simulink model "im_inv_model"  (R2026a)
settings: Solver=ode23tb  StopTime=param.sim.simlength  FixedStep=param.sim.tc  MaxStep=param.glb_time.tc  EnableMultiTasking=on
values from neighbouring files (symbols this model uses):
  param = struct()    [init_model.m]
undefined symbols (not defined in the file or in its folder): magnitude
libraries: fl_lib x53, nesl_utility x25, simulink x2, lithium_ion_battery x1, induction_machine x1, threephase_inductor_lib x1, dclink_with_center_tap x1, cstblocks_lti x1
(part 3 of 3)

== system im_inv_model/inverter//ctrl/im_ctrl/im_control/current control/bounder1 ==
  md : Inport
  k_sat : Inport  Port=2
  m : Inport  Port=3
  Constant : Constant
  Constant1 : Constant  Value=0
  Divide : Product
  Switch : Switch  Threshold=sqrt(3)/2  SaturateOnIntegerOverflow=off  InputSameDT=off
  Switch1 : Switch  Threshold=1 %sqrt(3)/2  SaturateOnIntegerOverflow=off  InputSameDT=off
  md_sat : Outport  VectorParamsAs1DForOutWhenUnconnected=off
  clip : Outport  Port=2  VectorParamsAs1DForOutWhenUnconnected=off
  wires:
  md/1 -> Switch1/3, Divide/2
  k_sat/1 -> Divide/1
  Divide/1 -> Switch1/1
  Switch1/1 -> md_sat/1
  Switch/1 -> clip/1
  m/1 -> Switch/2, Switch1/2
  Constant/1 -> Switch/1
  Constant1/1 -> Switch/3

== system im_inv_model/inverter//ctrl/im_ctrl/im_control/current control/bounder2 ==
  m : Inport
  k_sat : Inport  Port=2
  mq : Inport  Port=3
  Constant : Constant
  Constant1 : Constant  Value=0
  Divide : Product
  Switch : Switch  Threshold=sqrt(3)/2  SaturateOnIntegerOverflow=off  InputSameDT=off
  Switch1 : Switch  Threshold=1 %sqrt(3)/2  SaturateOnIntegerOverflow=off  InputSameDT=off
  mq_sat : Outport  VectorParamsAs1DForOutWhenUnconnected=off
  clip : Outport  Port=2  VectorParamsAs1DForOutWhenUnconnected=off
  wires:
  Constant1/1 -> Switch/3
  Constant/1 -> Switch/1
  m/1 -> Switch1/2, Switch/2
  Switch/1 -> clip/1
  Switch1/1 -> mq_sat/1
  Divide/1 -> Switch1/1
  k_sat/1 -> Divide/1
  mq/1 -> Divide/2, Switch1/3

== system im_inv_model/inverter//ctrl/im_ctrl/im_control/current control/pi-ctrl-x ==
  id_tilde : Inport
  clip : Inport  Port=2
  1/Ti : Gain  Gain=param.im.ctrl.kp_inv_d  SaturateOnIntegerOverflow=on  OutDataTypeStr=Inherit: Same as input  ParamDataTypeStr=Inherit: Same as input
  Constant : Constant  Value=0
  Sum2 : Sum  Inputs=+-  SaturateOnIntegerOverflow=on
  Sum4 : Sum  SaturateOnIntegerOverflow=on
  Sum5 : Sum  SaturateOnIntegerOverflow=on
  Switch1 : Switch  Threshold=0.5  SaturateOnIntegerOverflow=off  InputSameDT=off
  Switch2 : Switch  Threshold=0.5  SaturateOnIntegerOverflow=off  InputSameDT=off
  Unit Delay1 : UnitDelay  SampleTime=param.glb_time.ts_inv
  Unit Delay2 : UnitDelay  SampleTime=param.glb_time.ts_inv
  kp1 : Gain  Gain=param.ctrl.CTRPIFF_CLIP_RELEASE*param.glb_time.ts_inv  SaturateOnIntegerOverflow=on  OutDataTypeStr=Inherit: Same as input  ParamDataTypeStr=Inherit: Same as input
  kp2 : Gain  Gain=param.im.ctrl.ki_inv_d*param.glb_time.ts_inv  SaturateOnIntegerOverflow=on  OutDataTypeStr=Inherit: Same as input  ParamDataTypeStr=Inherit: Same as input
  Vds_out : Outport  VectorParamsAs1DForOutWhenUnconnected=off
  wires:
  id_tilde/1 -> kp2/1, 1/Ti/1
  Sum5/1 -> Vds_out/1
  Switch1/1 -> Unit Delay2/1
  Sum4/1 -> Sum5/2, Switch1/3
  kp1/1 -> Sum2/2
  Sum2/1 -> Switch1/1
  Unit Delay2/1 -> Sum4/2, kp1/1, Sum2/1
  1/Ti/1 -> Sum5/1
  Switch2/1 -> Sum4/1
  kp2/1 -> Switch2/3
  clip/1 -> Unit Delay1/1
  [clip] -> Switch2/2
  [clip] -> Switch1/2
  Constant/1 -> Switch2/1
  Unit Delay1/1 -> [clip]

== system im_inv_model/inverter//ctrl/im_ctrl/im_control/current control/pi-ctrl-y ==
  iq_tilde : Inport
  clip : Inport  Port=2
  1/Ti : Gain  Gain=param.im.ctrl.kp_inv_q  SaturateOnIntegerOverflow=on  OutDataTypeStr=Inherit: Same as input  ParamDataTypeStr=Inherit: Same as input
  Constant : Constant  Value=0
  Sum2 : Sum  Inputs=+-  SaturateOnIntegerOverflow=on
  Sum4 : Sum  SaturateOnIntegerOverflow=on
  Sum5 : Sum  SaturateOnIntegerOverflow=on
  Switch1 : Switch  Threshold=0.5  SaturateOnIntegerOverflow=off  InputSameDT=off
  Switch2 : Switch  Threshold=0.5  SaturateOnIntegerOverflow=off  InputSameDT=off
  Unit Delay1 : UnitDelay  SampleTime=param.glb_time.ts_inv
  Unit Delay2 : UnitDelay  SampleTime=param.glb_time.ts_inv
  kp1 : Gain  Gain=param.ctrl.CTRPIFF_CLIP_RELEASE*param.glb_time.ts_inv  SaturateOnIntegerOverflow=on  OutDataTypeStr=Inherit: Same as input  ParamDataTypeStr=Inherit: Same as input
  kp2 : Gain  Gain=param.im.ctrl.ki_inv_q*param.glb_time.ts_inv  SaturateOnIntegerOverflow=on  OutDataTypeStr=Inherit: Same as input  ParamDataTypeStr=Inherit: Same as input
  Vqs_out : Outport  VectorParamsAs1DForOutWhenUnconnected=off
  wires:
  Constant/1 -> Switch2/1
  [clip] -> Switch1/2
  [clip] -> Switch2/2
  clip/1 -> Unit Delay1/1
  kp2/1 -> Switch2/3
  Switch2/1 -> Sum4/1
  1/Ti/1 -> Sum5/1
  Unit Delay2/1 -> Sum2/1, kp1/1, Sum4/2
  Sum2/1 -> Switch1/1
  kp1/1 -> Sum2/2
  Sum4/1 -> Sum5/2, Switch1/3
  Switch1/1 -> Unit Delay2/1
  Sum5/1 -> Vqs_out/1
  iq_tilde/1 -> 1/Ti/1, kp2/1
  Unit Delay1/1 -> [clip]

== system im_inv_model/inverter//ctrl/im_ctrl/im_control/current control/switch ==
  clip 1 : Inport
  clip 2 : Inport  Port=2
  Constant4 : Constant
  Constant5 : Constant  Value=0
  Sum1 : Sum  SaturateOnIntegerOverflow=on
  Switch : Switch  Threshold=0.5  SaturateOnIntegerOverflow=off  InputSameDT=off
  clip : Outport  VectorParamsAs1DForOutWhenUnconnected=off
  wires:
  Constant5/1 -> Switch/3
  Switch/1 -> clip/1
  Constant4/1 -> Switch/1
  Sum1/1 -> Switch/2
  clip 1/1 -> Sum1/1
  clip 2/1 -> Sum1/2

== system im_inv_model/inverter//ctrl/im_ctrl/im_control/current control/vector lenght ==
  md : Inport
  mq : Inport  Port=2
  1/Ti3 : Gain  Gain=sqrt(3)/2  SaturateOnIntegerOverflow=on  OutDataTypeStr=Inherit: Same as input  ParamDataTypeStr=Inherit: Same as input
  Math Function : Math  Operator=magnitude^2  SignedPower=on
  Math Function1 : Math  Operator=magnitude^2  SignedPower=on
  Math Function2 : Math  Operator=reciprocal  SignedPower=on
  Sqrt : Sqrt
  Sum5 : Sum  SaturateOnIntegerOverflow=on
  k_sat : Outport  VectorParamsAs1DForOutWhenUnconnected=off
  m : Outport  Port=2  VectorParamsAs1DForOutWhenUnconnected=off
  wires:
  Sqrt/1 -> m/1, Math Function2/1
  mq/1 -> Math Function1/1
  Math Function1/1 -> Sum5/2
  Math Function/1 -> Sum5/1
  Sum5/1 -> Sqrt/1
  Math Function2/1 -> k_sat/1
  md/1 -> Math Function/1

== system im_inv_model/inverter//ctrl/im_ctrl/im_control/data_analysis/double_integrator_observer_1 ==
  theta : Inport
  Gain : Gain  Gain=param.im.ctrl.di_obs.komega
  Gain1 : Gain  Gain=param.im.ctrl.di_obs.ktheta
  Gain2 : Gain  Gain=param.im.machine.omega_bez
  Gain3 : Gain  Gain=1/param.im.machine.omega_bez
  Gain5 : Gain  Gain=param.glb_time.ts_inv
  Sum : Sum  Inputs=-+|
  Sum1 : Sum  Inputs=|++
  Sum2 : Sum  Inputs=|++
  Sum8 : Sum  Inputs=++|
  Unit Delay1 : UnitDelay  InitialCondition=pi  SampleTime=param.glb_time.ts_inv
  Unit Delay2 : UnitDelay  SampleTime=param.glb_time.ts_inv
  bounder1 : MATLAB Function  TreatAsAtomicUnit=on  SystemSampleTime=param.glb_time.ts_inv
  bounder2 : MATLAB Function  TreatAsAtomicUnit=on  SystemSampleTime=param.glb_time.ts_inv
  omega_pu_hat : Outport  VectorParamsAs1DForOutWhenUnconnected=off
  wires:
  Gain1/1 -> Sum2/1
  theta/1 -> Sum/2  "theta_bemf"
  Sum8/1 -> Unit Delay1/1
  Unit Delay1/1 -> bounder2/1(u)
  Sum1/1 -> Unit Delay2/1
  Gain/1 -> Gain3/1
  Unit Delay2/1 -> omega_pu_hat/1, Sum1/2, Gain5/1
  Sum2/1 -> Sum8/2
  bounder2/1(y) -> Sum2/2, Sum/1  "theta_hat"
  bounder1/1(y) -> Gain1/1, Gain/1
  Gain2/1 -> Sum8/1
  Gain3/1 -> Sum1/1
  Gain5/1 -> Gain2/1
  Sum/1 -> bounder1/1(u)

== system im_inv_model/inverter//ctrl/im_ctrl/im_control/data_analysis/double_integrator_observer_2 ==
  theta : Inport
  Gain : Gain  Gain=param.im.ctrl.di_obs.komega
  Gain1 : Gain  Gain=param.im.ctrl.di_obs.ktheta
  Gain2 : Gain  Gain=param.im.machine.omega_bez
  Gain3 : Gain  Gain=1/param.im.machine.omega_bez
  Gain5 : Gain  Gain=param.glb_time.ts_inv
  Sum : Sum  Inputs=-+|
  Sum1 : Sum  Inputs=|++
  Sum2 : Sum  Inputs=|++
  Sum8 : Sum  Inputs=++|
  Unit Delay1 : UnitDelay  InitialCondition=pi  SampleTime=param.glb_time.ts_inv
  Unit Delay2 : UnitDelay  SampleTime=param.glb_time.ts_inv
  bounder1 : MATLAB Function  TreatAsAtomicUnit=on  SystemSampleTime=param.glb_time.ts_inv
  bounder2 : MATLAB Function  TreatAsAtomicUnit=on  SystemSampleTime=param.glb_time.ts_inv
  omega_pu_hat : Outport  VectorParamsAs1DForOutWhenUnconnected=off
  wires:
  Sum/1 -> bounder1/1(u)
  Gain5/1 -> Gain2/1
  Gain3/1 -> Sum1/1
  Gain2/1 -> Sum8/1
  bounder1/1(y) -> Gain/1, Gain1/1
  bounder2/1(y) -> Sum/1, Sum2/2  "theta_hat"
  Sum2/1 -> Sum8/2
  Unit Delay2/1 -> Gain5/1, Sum1/2, omega_pu_hat/1
  Gain/1 -> Gain3/1
  Sum1/1 -> Unit Delay2/1
  Unit Delay1/1 -> bounder2/1(u)
  Sum8/1 -> Unit Delay1/1
  theta/1 -> Sum/2  "theta_bemf"
  Gain1/1 -> Sum2/1

== system im_inv_model/inverter//ctrl/im_ctrl/im_control/data_analysis/double_integrator_observer_3 ==
  theta : Inport
  Gain : Gain  Gain=param.im.ctrl.di_obs.komega
  Gain1 : Gain  Gain=param.im.ctrl.di_obs.ktheta
  Gain2 : Gain  Gain=param.im.machine.omega_bez
  Gain3 : Gain  Gain=1/param.im.machine.omega_bez
  Gain5 : Gain  Gain=param.glb_time.ts_inv
  Sum : Sum  Inputs=-+|
  Sum1 : Sum  Inputs=|++
  Sum2 : Sum  Inputs=|++
  Sum8 : Sum  Inputs=++|
  Unit Delay1 : UnitDelay  InitialCondition=pi  SampleTime=param.glb_time.ts_inv
  Unit Delay2 : UnitDelay  SampleTime=param.glb_time.ts_inv
  bounder1 : MATLAB Function  TreatAsAtomicUnit=on  SystemSampleTime=param.glb_time.ts_inv
  bounder2 : MATLAB Function  TreatAsAtomicUnit=on  SystemSampleTime=param.glb_time.ts_inv
  omega_pu_hat : Outport  VectorParamsAs1DForOutWhenUnconnected=off
  wires:
  Gain1/1 -> Sum2/1
  theta/1 -> Sum/2  "theta_bemf"
  Sum8/1 -> Unit Delay1/1
  Unit Delay1/1 -> bounder2/1(u)
  Sum1/1 -> Unit Delay2/1
  Gain/1 -> Gain3/1
  Unit Delay2/1 -> omega_pu_hat/1, Sum1/2, Gain5/1
  Sum2/1 -> Sum8/2
  bounder2/1(y) -> Sum2/2, Sum/1  "theta_hat"
  bounder1/1(y) -> Gain1/1, Gain/1
  Gain2/1 -> Sum8/1
  Gain3/1 -> Sum1/1
  Gain5/1 -> Gain2/1
  Sum/1 -> bounder1/1(u)

== system im_inv_model/inverter//ctrl/im_ctrl/im_control/flux_estimator/alphabeta2dq ==
  alpha : Inport
  beta : Inport  Port=2
  phase : Inport  Port=3
  Gain : Gain
  Gain1 : Gain
  Product{,1..3} (4 alike) : Product  RndMeth=Zero
  Sum : Sum
  Sum1 : Sum  Inputs=-+
  Trigonometric Function : Trigonometry  Operator=cos
  Trigonometric Function1 : Trigonometry
  d : Outport  VectorParamsAs1DForOutWhenUnconnected=off
  q : Outport  Port=2  VectorParamsAs1DForOutWhenUnconnected=off
  wires:
  [cos] -> Product/1
  alpha/1 -> Product/2, Product2/2
  Product/1 -> Sum/1
  Product1/1 -> Sum/2
  [sin] -> Product1/1
  beta/1 -> Product1/2, Product3/2
  Sum/1 -> Gain/1
  [sin] -> Product2/1
  Product2/1 -> Sum1/1
  Product3/1 -> Sum1/2
  [cos] -> Product3/1
  Sum1/1 -> Gain1/1
  Gain/1 -> d/1
  Gain1/1 -> q/1
  Trigonometric Function1/1 -> [sin]
  Trigonometric Function/1 -> [cos]
  phase/1 -> Trigonometric Function/1, Trigonometric Function1/1

== system im_inv_model/inverter//ctrl/im_ctrl/im_control/magnetization current reference/pi ==
  psi_r_hat : Inport
  psi_r_ref : Inport  Port=2
  1/Ti : Gain  Gain=param.im.ctrl.kp_psi  SaturateOnIntegerOverflow=on  OutDataTypeStr=Inherit: Same as input  ParamDataTypeStr=Inherit: Same as input
  Saturation : Saturate  UpperLimit=param.im.ctrl.isx_lim_max*param.im.machine.Lm_norm  LowerLimit=param.im.ctrl.isx_lim_min*param.im.machine.Lm_norm
  Sum1 : Sum  Inputs=+++  SaturateOnIntegerOverflow=on
  Sum2 : Sum  Inputs=-+  SaturateOnIntegerOverflow=on
  Sum3 : Sum  Inputs=-+  SaturateOnIntegerOverflow=on
  Unit Delay4 : UnitDelay  SampleTime=param.glb_time.ts_inv
  kp : Gain  Gain=param.im.ctrl.ki_psi*param.glb_time.ts_inv  SaturateOnIntegerOverflow=on  OutDataTypeStr=Inherit: Same as input  ParamDataTypeStr=Inherit: Same as input
  psi_s_ref : Outport  VectorParamsAs1DForOutWhenUnconnected=off
  wires:
  1/Ti/1 -> Sum1/1, Sum3/1
  kp/1 -> Sum1/2
  Sum2/1 -> 1/Ti/1, kp/1
  Sum1/1 -> Saturation/1
  Sum3/1 -> Unit Delay4/1
  Unit Delay4/1 -> Sum1/3
  psi_r_ref/1 -> Sum2/2
  psi_r_hat/1 -> Sum2/1
  Saturation/1 -> psi_s_ref/1, Sum3/2

== system im_inv_model/inverter//ctrl/im_ctrl/im_control/u//f control/uf_phase_generation ==
  Constant1 : Constant  Value=param.im.uf.omega_ref
  Gain : Gain  Gain=param.im.uf.Omega_s_bez
  Integrator : Integrator
  Zero-Order Hold : ZeroOrderHold  SampleTime=param.glb_time.ts_inv
  bounder : MATLAB Function  TreatAsAtomicUnit=on  SystemSampleTime=param.glb_time.ts_inv
  uf_electrical_phase : Outport
  wires:
  Gain/1 -> Integrator/1
  Integrator/1 -> Zero-Order Hold/1
  Zero-Order Hold/1 -> bounder/1(u)
  Constant1/1 -> Gain/1
  bounder/1(y) -> uf_electrical_phase/1

== system im_inv_model/inverter//ctrl/inverter/inverter/sv_pwm/modulator1 ==
  u : Inport
  v : Inport  Port=2
  w : Inport  Port=3
  phase : Inport  Port=4
  Bus Creator3 : BusCreator  Inputs=6
  PWM generator 1 : Subsystem  mask{f=param.glb_time.fPWM_INV, m_up=0.98, m_low=0.02, dead_time=param.glb_time.dead_time_INV, pos_cmd_gate=15, neg_cmd_gate=-10, polarity=-1}
      mask prompts: f "Frequency (Hz)"; m_up "Max Input Modulation Value"; m_low "Min Input Modulation Value"; dead_time "Dead Time (s)"; pos_cmd_gate "Positive Gate Voltage (V)"; neg_cmd_gate "Negative Gate Voltage (V)"; polarity "Polarity (pu)"
  PWM generator 2 : Subsystem  mask{f=param.glb_time.fPWM_INV, m_up=0.98, m_low=0.02, dead_time=param.glb_time.dead_time_INV, pos_cmd_gate=15, neg_cmd_gate=-10, polarity=-1}
      mask prompts: f "Frequency (Hz)"; m_up "Max Input Modulation Value"; m_low "Min Input Modulation Value"; dead_time "Dead Time (s)"; pos_cmd_gate "Positive Gate Voltage (V)"; neg_cmd_gate "Negative Gate Voltage (V)"; polarity "Polarity (pu)"
  PWM generator 3 : Subsystem  mask{f=param.glb_time.fPWM_INV, m_up=0.98, m_low=0.02, dead_time=param.glb_time.dead_time_INV, pos_cmd_gate=15, neg_cmd_gate=-10, polarity=-1}
      mask prompts: f "Frequency (Hz)"; m_up "Max Input Modulation Value"; m_low "Min Input Modulation Value"; dead_time "Dead Time (s)"; pos_cmd_gate "Positive Gate Voltage (V)"; neg_cmd_gate "Negative Gate Voltage (V)"; polarity "Polarity (pu)"
  cmd_gates : Outport
  wires:
  u/1 -> PWM generator 1/1(m_index)
  w/1 -> PWM generator 3/1(m_index)
  v/1 -> PWM generator 2/1(m_index)
  phase/1 -> PWM generator 3/2(phase), PWM generator 2/2(phase), PWM generator 1/2(phase)
  PWM generator 1/2(m2) -> Bus Creator3/2  "gate_cmd_Q2"
  PWM generator 3/1(m1) -> Bus Creator3/5  "gate_cmd_Q5"
  PWM generator 2/1(m1) -> Bus Creator3/3  "gate_cmd_Q3"
  PWM generator 2/2(m2) -> Bus Creator3/4  "gate_cmd_Q4"
  PWM generator 3/2(m2) -> Bus Creator3/6  "gate_cmd_Q6"
  PWM generator 1/1(m1) -> Bus Creator3/1  "gate_cmd_Q1"
  Bus Creator3/1 -> cmd_gates/1

== system im_inv_model/inverter//ctrl/inverter/inverter/three phase pwm/Third harmonic injecting ==
  m1 : Inport
  m2 : Inport  Port=2
  m3 : Inport  Port=3
  Gain : Gain  Gain=1/2
  MinMax : MinMax  Function=max  Inputs=3
  MinMax1 : MinMax  Inputs=3
  Sum : Sum  Inputs=|++
  trn : Outport
  wires:
  Gain/1 -> trn/1
  Sum/1 -> Gain/1
  MinMax1/1 -> Sum/2
  MinMax/1 -> Sum/1
  m3/1 -> MinMax/3, MinMax1/3
  m1/1 -> MinMax1/1, MinMax/1
  m2/1 -> MinMax1/2, MinMax/2

== system im_inv_model/inverter//ctrl/inverter/inverter/three phase pwm/modulator ==
  u : Inport
  v : Inport  Port=2
  w : Inport  Port=3
  phase : Inport  Port=4
  Bus Creator3 : BusCreator  Inputs=6
  PWM generator 1 : Subsystem  mask{f=param.glb_time.fPWM_INV, m_up=1, m_low=0, dead_time=0, vg_firing=15}
      mask prompts: f "Frequency"; m_up "Max Input Modulation Value"; m_low "Min Input Modulation Value"; dead_time "Dead Time"; vg_firing "Gate Voltage"
  PWM generator 2 : Subsystem  mask{f=param.glb_time.fPWM_INV, m_up=1, m_low=0, dead_time=0, vg_firing=15}
      mask prompts: f "Frequency"; m_up "Max Input Modulation Value"; m_low "Min Input Modulation Value"; dead_time "Dead Time"; vg_firing "Gate Voltage"
  PWM generator 3 : Subsystem  mask{f=param.glb_time.fPWM_INV, m_up=1, m_low=0, dead_time=0, vg_firing=15}
      mask prompts: f "Frequency"; m_up "Max Input Modulation Value"; m_low "Min Input Modulation Value"; dead_time "Dead Time"; vg_firing "Gate Voltage"
  cmd_gates : Outport
  wires:
  u/1 -> PWM generator 1/1(m_index)
  w/1 -> PWM generator 3/1(m_index)
  v/1 -> PWM generator 2/1(m_index)
  phase/1 -> PWM generator 3/2(phase), PWM generator 2/2(phase), PWM generator 1/2(phase)
  PWM generator 3/2(m2) -> Bus Creator3/6  "gate_cmd_Q6"
  Bus Creator3/1 -> cmd_gates/1
  PWM generator 2/2(m2) -> Bus Creator3/4  "gate_cmd_Q4"
  PWM generator 1/1(m1) -> Bus Creator3/1  "gate_cmd_Q1"
  PWM generator 3/1(m1) -> Bus Creator3/5  "gate_cmd_Q5"
  PWM generator 1/2(m2) -> Bus Creator3/2  "gate_cmd_Q2"
  PWM generator 2/1(m1) -> Bus Creator3/3  "gate_cmd_Q3"

== system im_inv_model/inverter//ctrl/inverter/inverter/three phase pwm1/PWM generator 1 ==
  m_index : Inport
  Constant : Constant  Value=dead_time*f*2
  Data Type Conversion1 : DataTypeConversion
  Data Type Conversion2 : DataTypeConversion
  Gain : Gain  Gain=1/(pi/2)
  Gain1 : Gain  Gain=sqrt(3)/2
  Hit Crossing : HitCross  ShowOutputPort=off
  Hit Crossing1 : HitCross  ShowOutputPort=off
  Relational Operator1 : RelationalOperator  Operator=<=  InputSameDT=off
  Relational Operator2 : RelationalOperator  Operator=<=  InputSameDT=off
  Saturation1 : Saturate  UpperLimit=m_up  LowerLimit=m_low
  Sine Wave : Sin  Frequency=f*2*pi  Phase=-pi/2+ph  SampleTime=0
  Sum : Sum  Inputs=|++  SaturateOnIntegerOverflow=on
  Sum1 : Sum  Inputs=-+|  SaturateOnIntegerOverflow=on
  Trigonometric Function1 : Trigonometry  Operator=asin
  m1 : Outport
  m2 : Outport  Port=2
  wires:
  Relational Operator1/1 -> Data Type Conversion1/1
  m_index/1 -> Saturation1/1
  Data Type Conversion1/1 -> Hit Crossing/1, m2/1
  Relational Operator2/1 -> Data Type Conversion2/1
  Data Type Conversion2/1 -> Hit Crossing1/1, m1/1
  Constant/1 -> Sum/2, Sum1/1
  Saturation1/1 -> Sum/1, Sum1/2
  Sum/1 -> Relational Operator1/1
  Sum1/1 -> Relational Operator2/2
  Sine Wave/1 -> Trigonometric Function1/1
  Trigonometric Function1/1 -> Gain/1
  Gain/1 -> Gain1/1
  Gain1/1 -> Relational Operator1/2, Relational Operator2/1

== system im_inv_model/inverter//ctrl/inverter/inverter/three phase pwm1/PWM generator 2 ==
  m_index : Inport
  Constant : Constant  Value=dead_time*f*2
  Data Type Conversion1 : DataTypeConversion
  Data Type Conversion2 : DataTypeConversion
  Gain : Gain  Gain=1/(pi/2)
  Gain1 : Gain  Gain=sqrt(3)/2
  Hit Crossing : HitCross  ShowOutputPort=off
  Hit Crossing1 : HitCross  ShowOutputPort=off
  Relational Operator1 : RelationalOperator  Operator=<=  InputSameDT=off
  Relational Operator2 : RelationalOperator  Operator=<=  InputSameDT=off
  Saturation1 : Saturate  UpperLimit=m_up  LowerLimit=m_low
  Sine Wave : Sin  Frequency=f*2*pi  Phase=-pi/2+ph  SampleTime=0
  Sum : Sum  Inputs=|++  SaturateOnIntegerOverflow=on
  Sum1 : Sum  Inputs=-+|  SaturateOnIntegerOverflow=on
  Trigonometric Function1 : Trigonometry  Operator=asin
  m1 : Outport
  m2 : Outport  Port=2
  wires:
  Gain1/1 -> Relational Operator2/1, Relational Operator1/2
  Gain/1 -> Gain1/1
  Trigonometric Function1/1 -> Gain/1
  Sine Wave/1 -> Trigonometric Function1/1
  Sum1/1 -> Relational Operator2/2
  Sum/1 -> Relational Operator1/1
  Saturation1/1 -> Sum1/2, Sum/1
  Constant/1 -> Sum1/1, Sum/2
  Data Type Conversion2/1 -> m1/1, Hit Crossing1/1
  Relational Operator2/1 -> Data Type Conversion2/1
  Data Type Conversion1/1 -> m2/1, Hit Crossing/1
  m_index/1 -> Saturation1/1
  Relational Operator1/1 -> Data Type Conversion1/1

== system im_inv_model/inverter//ctrl/inverter/inverter/three phase pwm1/PWM generator 3 ==
  m_index : Inport
  Constant : Constant  Value=dead_time*f*2
  Data Type Conversion1 : DataTypeConversion
  Data Type Conversion2 : DataTypeConversion
  Gain : Gain  Gain=1/(pi/2)
  Gain1 : Gain  Gain=sqrt(3)/2
  Hit Crossing : HitCross  ShowOutputPort=off
  Hit Crossing1 : HitCross  ShowOutputPort=off
  Relational Operator1 : RelationalOperator  Operator=<=  InputSameDT=off
  Relational Operator2 : RelationalOperator  Operator=<=  InputSameDT=off
  Saturation1 : Saturate  UpperLimit=m_up  LowerLimit=m_low
  Sine Wave : Sin  Frequency=f*2*pi  Phase=-pi/2+ph  SampleTime=0
  Sum : Sum  Inputs=|++  SaturateOnIntegerOverflow=on
  Sum1 : Sum  Inputs=-+|  SaturateOnIntegerOverflow=on
  Trigonometric Function1 : Trigonometry  Operator=asin
  m1 : Outport
  m2 : Outport  Port=2
  wires:
  Relational Operator1/1 -> Data Type Conversion1/1
  m_index/1 -> Saturation1/1
  Data Type Conversion1/1 -> Hit Crossing/1, m2/1
  Relational Operator2/1 -> Data Type Conversion2/1
  Data Type Conversion2/1 -> Hit Crossing1/1, m1/1
  Constant/1 -> Sum/2, Sum1/1
  Saturation1/1 -> Sum/1, Sum1/2
  Sum/1 -> Relational Operator1/1
  Sum1/1 -> Relational Operator2/2
  Sine Wave/1 -> Trigonometric Function1/1
  Trigonometric Function1/1 -> Gain/1
  Gain/1 -> Gain1/1
  Gain1/1 -> Relational Operator1/2, Relational Operator2/1

== system im_inv_model/inverter//ctrl/inverter/inverter/three phase pwm1/Third harmonic injecting ==
  m1 : Inport
  m2 : Inport  Port=2
  m3 : Inport  Port=3
  Gain : Gain  Gain=1/2
  MinMax : MinMax  Function=max  Inputs=3
  MinMax1 : MinMax  Inputs=3
  Sum : Sum  Inputs=|++
  thind_H : Outport
  wires:
  m2/1 -> MinMax/2, MinMax1/2
  m1/1 -> MinMax/1, MinMax1/1
  m3/1 -> MinMax/3, MinMax1/3
  MinMax/1 -> Sum/1
  MinMax1/1 -> Sum/2
  Sum/1 -> Gain/1
  Gain/1 -> thind_H/1

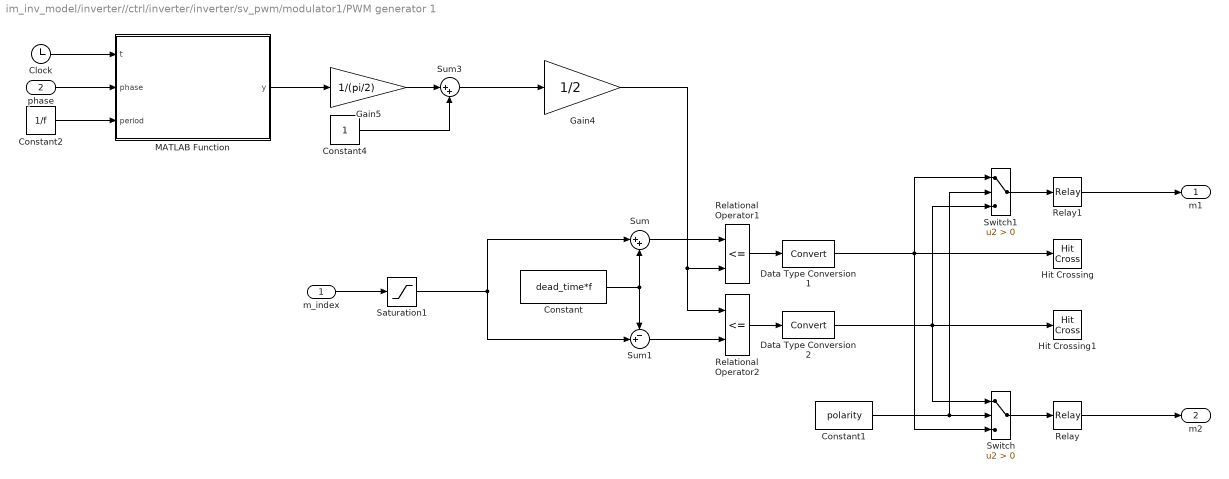
== system im_inv_model/inverter//ctrl/inverter/inverter/sv_pwm/modulator1/PWM generator 1 ==
  m_index : Inport
  phase : Inport  Port=2
  Clock : Clock
  Constant : Constant  Value=dead_time*f
  Constant1 : Constant  Value=polarity
  Constant2 : Constant  Value=1/f
  Constant4 : Constant
  Data Type Conversion1 : DataTypeConversion
  Data Type Conversion2 : DataTypeConversion
  Gain4 : Gain  Gain=1/2
  Gain5 : Gain  Gain=1/(pi/2)
  Hit Crossing : HitCross  ShowOutputPort=off
  Hit Crossing1 : HitCross  ShowOutputPort=off
  MATLAB Function : MATLAB Function  TreatAsAtomicUnit=on
  Relational Operator1 : RelationalOperator  Operator=<=  InputSameDT=off
  Relational Operator2 : RelationalOperator  Operator=<=  InputSameDT=off
  Relay : Relay  OnOutputValue=pos_cmd_gate  OffOutputValue=neg_cmd_gate
  Relay1 : Relay  OnOutputValue=pos_cmd_gate  OffOutputValue=neg_cmd_gate
  Saturation1 : Saturate  UpperLimit=m_up  LowerLimit=m_low
  Sum : Sum  Inputs=|++  SaturateOnIntegerOverflow=on
  Sum1 : Sum  Inputs=-+|  SaturateOnIntegerOverflow=on
  Sum3 : Sum  Inputs=|++
  Switch : Switch  Criteria=u2 > Threshold  SaturateOnIntegerOverflow=off  InputSameDT=off
  Switch1 : Switch  Criteria=u2 > Threshold  SaturateOnIntegerOverflow=off  InputSameDT=off
  m1 : Outport
  m2 : Outport  Port=2
  wires:
  Relational Operator1/1 -> Data Type Conversion1/1
  m_index/1 -> Saturation1/1
  Relational Operator2/1 -> Data Type Conversion2/1
  Data Type Conversion2/1 -> Switch/1, Switch1/3, Hit Crossing1/1
  Constant/1 -> Sum/2, Sum1/1
  Saturation1/1 -> Sum/1, Sum1/2
  Sum/1 -> Relational Operator1/1
  Sum1/1 -> Relational Operator2/2
  Gain4/1 -> Relational Operator2/1, Relational Operator1/2
  Data Type Conversion1/1 -> Hit Crossing/1, Switch/3, Switch1/1
  Switch/1 -> Relay/1
  Clock/1 -> MATLAB Function/1(t)
  Constant2/1 -> MATLAB Function/3(period)
  phase/1 -> MATLAB Function/2(phase)
  MATLAB Function/1(y) -> Gain5/1
  Gain5/1 -> Sum3/1
  Sum3/1 -> Gain4/1
  Constant4/1 -> Sum3/2
  Relay/1 -> m2/1
  Constant1/1 -> Switch1/2, Switch/2
  Switch1/1 -> Relay1/1
  Relay1/1 -> m1/1

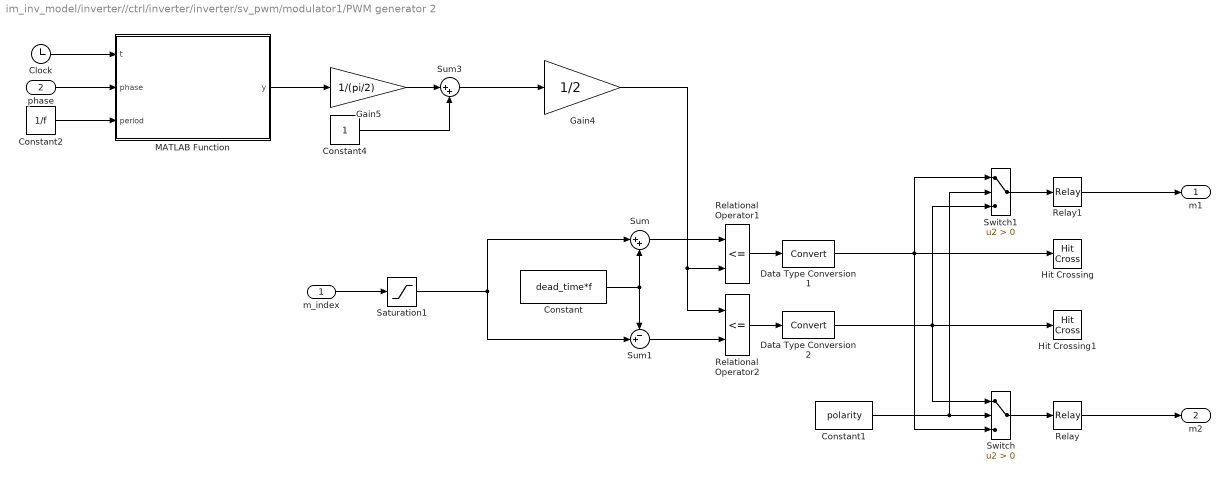
== system im_inv_model/inverter//ctrl/inverter/inverter/sv_pwm/modulator1/PWM generator 2 ==
  m_index : Inport
  phase : Inport  Port=2
  Clock : Clock
  Constant : Constant  Value=dead_time*f
  Constant1 : Constant  Value=polarity
  Constant2 : Constant  Value=1/f
  Constant4 : Constant
  Data Type Conversion1 : DataTypeConversion
  Data Type Conversion2 : DataTypeConversion
  Gain4 : Gain  Gain=1/2
  Gain5 : Gain  Gain=1/(pi/2)
  Hit Crossing : HitCross  ShowOutputPort=off
  Hit Crossing1 : HitCross  ShowOutputPort=off
  MATLAB Function : MATLAB Function  TreatAsAtomicUnit=on
  Relational Operator1 : RelationalOperator  Operator=<=  InputSameDT=off
  Relational Operator2 : RelationalOperator  Operator=<=  InputSameDT=off
  Relay : Relay  OnOutputValue=pos_cmd_gate  OffOutputValue=neg_cmd_gate
  Relay1 : Relay  OnOutputValue=pos_cmd_gate  OffOutputValue=neg_cmd_gate
  Saturation1 : Saturate  UpperLimit=m_up  LowerLimit=m_low
  Sum : Sum  Inputs=|++  SaturateOnIntegerOverflow=on
  Sum1 : Sum  Inputs=-+|  SaturateOnIntegerOverflow=on
  Sum3 : Sum  Inputs=|++
  Switch : Switch  Criteria=u2 > Threshold  SaturateOnIntegerOverflow=off  InputSameDT=off
  Switch1 : Switch  Criteria=u2 > Threshold  SaturateOnIntegerOverflow=off  InputSameDT=off
  m1 : Outport
  m2 : Outport  Port=2
  wires:
  Relay1/1 -> m1/1
  Switch1/1 -> Relay1/1
  Constant1/1 -> Switch/2, Switch1/2
  Relay/1 -> m2/1
  Constant4/1 -> Sum3/2
  Sum3/1 -> Gain4/1
  Gain5/1 -> Sum3/1
  MATLAB Function/1(y) -> Gain5/1
  phase/1 -> MATLAB Function/2(phase)
  Constant2/1 -> MATLAB Function/3(period)
  Clock/1 -> MATLAB Function/1(t)
  Switch/1 -> Relay/1
  Data Type Conversion1/1 -> Switch1/1, Switch/3, Hit Crossing/1
  Gain4/1 -> Relational Operator1/2, Relational Operator2/1
  Sum1/1 -> Relational Operator2/2
  Sum/1 -> Relational Operator1/1
  Saturation1/1 -> Sum1/2, Sum/1
  Constant/1 -> Sum1/1, Sum/2
  Data Type Conversion2/1 -> Hit Crossing1/1, Switch1/3, Switch/1
  Relational Operator2/1 -> Data Type Conversion2/1
  m_index/1 -> Saturation1/1
  Relational Operator1/1 -> Data Type Conversion1/1

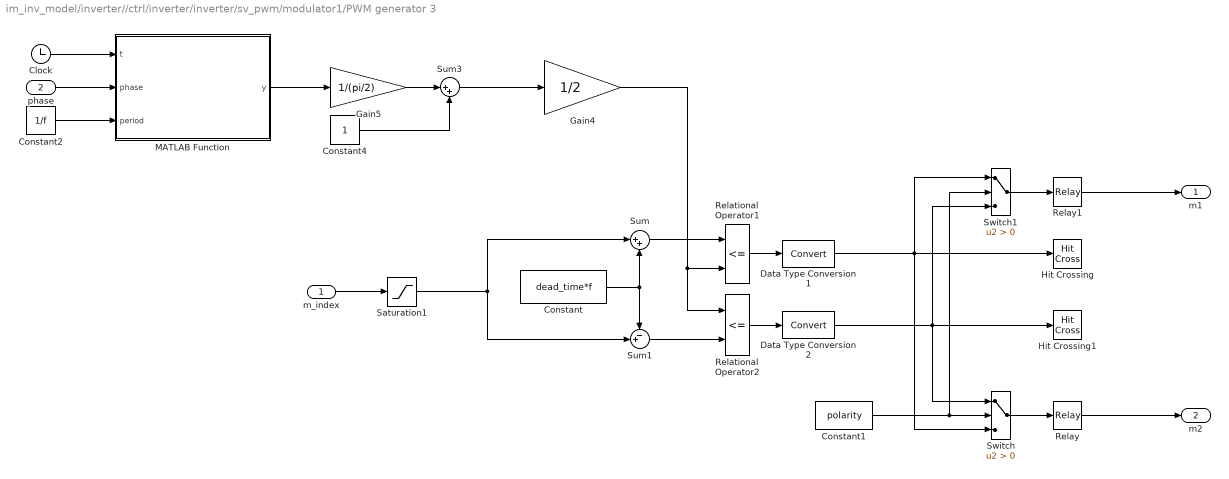
== system im_inv_model/inverter//ctrl/inverter/inverter/sv_pwm/modulator1/PWM generator 3 ==
  m_index : Inport
  phase : Inport  Port=2
  Clock : Clock
  Constant : Constant  Value=dead_time*f
  Constant1 : Constant  Value=polarity
  Constant2 : Constant  Value=1/f
  Constant4 : Constant
  Data Type Conversion1 : DataTypeConversion
  Data Type Conversion2 : DataTypeConversion
  Gain4 : Gain  Gain=1/2
  Gain5 : Gain  Gain=1/(pi/2)
  Hit Crossing : HitCross  ShowOutputPort=off
  Hit Crossing1 : HitCross  ShowOutputPort=off
  MATLAB Function : MATLAB Function  TreatAsAtomicUnit=on
  Relational Operator1 : RelationalOperator  Operator=<=  InputSameDT=off
  Relational Operator2 : RelationalOperator  Operator=<=  InputSameDT=off
  Relay : Relay  OnOutputValue=pos_cmd_gate  OffOutputValue=neg_cmd_gate
  Relay1 : Relay  OnOutputValue=pos_cmd_gate  OffOutputValue=neg_cmd_gate
  Saturation1 : Saturate  UpperLimit=m_up  LowerLimit=m_low
  Sum : Sum  Inputs=|++  SaturateOnIntegerOverflow=on
  Sum1 : Sum  Inputs=-+|  SaturateOnIntegerOverflow=on
  Sum3 : Sum  Inputs=|++
  Switch : Switch  Criteria=u2 > Threshold  SaturateOnIntegerOverflow=off  InputSameDT=off
  Switch1 : Switch  Criteria=u2 > Threshold  SaturateOnIntegerOverflow=off  InputSameDT=off
  m1 : Outport
  m2 : Outport  Port=2
  wires:
  Relational Operator1/1 -> Data Type Conversion1/1
  m_index/1 -> Saturation1/1
  Relational Operator2/1 -> Data Type Conversion2/1
  Data Type Conversion2/1 -> Switch/1, Switch1/3, Hit Crossing1/1
  Constant/1 -> Sum/2, Sum1/1
  Saturation1/1 -> Sum/1, Sum1/2
  Sum/1 -> Relational Operator1/1
  Sum1/1 -> Relational Operator2/2
  Gain4/1 -> Relational Operator2/1, Relational Operator1/2
  Data Type Conversion1/1 -> Hit Crossing/1, Switch/3, Switch1/1
  Switch/1 -> Relay/1
  Clock/1 -> MATLAB Function/1(t)
  Constant2/1 -> MATLAB Function/3(period)
  phase/1 -> MATLAB Function/2(phase)
  MATLAB Function/1(y) -> Gain5/1
  Gain5/1 -> Sum3/1
  Sum3/1 -> Gain4/1
  Constant4/1 -> Sum3/2
  Relay/1 -> m2/1
  Constant1/1 -> Switch1/2, Switch/2
  Switch1/1 -> Relay1/1
  Relay1/1 -> m1/1

== system im_inv_model/inverter//ctrl/inverter/inverter/three phase pwm/modulator/PWM generator 1 ==
  m_index : Inport
  phase : Inport  Port=2
  Clock : Clock
  Constant : Constant  Value=dead_time*f
  Constant2 : Constant  Value=1/f
  Constant4 : Constant
  Data Type Conversion1 : DataTypeConversion
  Data Type Conversion2 : DataTypeConversion
  Gain2 : Gain  Gain=vg_firing
  Gain3 : Gain  Gain=vg_firing
  Gain4 : Gain  Gain=1/2
  Gain5 : Gain  Gain=1/(pi/2)
  Hit Crossing : HitCross  ShowOutputPort=off
  Hit Crossing1 : HitCross  ShowOutputPort=off
  MATLAB Function : MATLAB Function  TreatAsAtomicUnit=on
  Relational Operator1 : RelationalOperator  Operator=<=  InputSameDT=off
  Relational Operator2 : RelationalOperator  Operator=<=  InputSameDT=off
  Saturation1 : Saturate  UpperLimit=m_up  LowerLimit=m_low
  Sum : Sum  Inputs=|++  SaturateOnIntegerOverflow=on
  Sum1 : Sum  Inputs=-+|  SaturateOnIntegerOverflow=on
  Sum3 : Sum  Inputs=|++
  m1 : Outport
  m2 : Outport  Port=2
  wires:
  Relational Operator1/1 -> Data Type Conversion1/1
  m_index/1 -> Saturation1/1
  Relational Operator2/1 -> Data Type Conversion2/1
  Data Type Conversion2/1 -> Gain3/1, Hit Crossing1/1
  Constant/1 -> Sum/2, Sum1/1
  Saturation1/1 -> Sum/1, Sum1/2
  Sum/1 -> Relational Operator1/1
  Sum1/1 -> Relational Operator2/2
  Gain4/1 -> Relational Operator2/1, Relational Operator1/2
  Data Type Conversion1/1 -> Hit Crossing/1, Gain2/1
  Gain2/1 -> m1/1
  Gain3/1 -> m2/1
  Clock/1 -> MATLAB Function/1(t)
  Constant2/1 -> MATLAB Function/3(period)
  phase/1 -> MATLAB Function/2(phase)
  MATLAB Function/1(y) -> Gain5/1
  Gain5/1 -> Sum3/1
  Sum3/1 -> Gain4/1
  Constant4/1 -> Sum3/2

== system im_inv_model/inverter//ctrl/inverter/inverter/three phase pwm/modulator/PWM generator 2 ==
  m_index : Inport
  phase : Inport  Port=2
  Clock : Clock
  Constant : Constant  Value=dead_time*f
  Constant2 : Constant  Value=1/f
  Constant4 : Constant
  Data Type Conversion1 : DataTypeConversion
  Data Type Conversion2 : DataTypeConversion
  Gain2 : Gain  Gain=vg_firing
  Gain3 : Gain  Gain=vg_firing
  Gain4 : Gain  Gain=1/2
  Gain5 : Gain  Gain=1/(pi/2)
  Hit Crossing : HitCross  ShowOutputPort=off
  Hit Crossing1 : HitCross  ShowOutputPort=off
  MATLAB Function : MATLAB Function  TreatAsAtomicUnit=on
  Relational Operator1 : RelationalOperator  Operator=<=  InputSameDT=off
  Relational Operator2 : RelationalOperator  Operator=<=  InputSameDT=off
  Saturation1 : Saturate  UpperLimit=m_up  LowerLimit=m_low
  Sum : Sum  Inputs=|++  SaturateOnIntegerOverflow=on
  Sum1 : Sum  Inputs=-+|  SaturateOnIntegerOverflow=on
  Sum3 : Sum  Inputs=|++
  m1 : Outport
  m2 : Outport  Port=2
  wires:
  Constant4/1 -> Sum3/2
  Sum3/1 -> Gain4/1
  Gain5/1 -> Sum3/1
  MATLAB Function/1(y) -> Gain5/1
  phase/1 -> MATLAB Function/2(phase)
  Constant2/1 -> MATLAB Function/3(period)
  Clock/1 -> MATLAB Function/1(t)
  Gain3/1 -> m2/1
  Gain2/1 -> m1/1
  Data Type Conversion1/1 -> Gain2/1, Hit Crossing/1
  Gain4/1 -> Relational Operator1/2, Relational Operator2/1
  Sum1/1 -> Relational Operator2/2
  Sum/1 -> Relational Operator1/1
  Saturation1/1 -> Sum1/2, Sum/1
  Constant/1 -> Sum1/1, Sum/2
  Data Type Conversion2/1 -> Hit Crossing1/1, Gain3/1
  Relational Operator2/1 -> Data Type Conversion2/1
  m_index/1 -> Saturation1/1
  Relational Operator1/1 -> Data Type Conversion1/1

== system im_inv_model/inverter//ctrl/inverter/inverter/three phase pwm/modulator/PWM generator 3 ==
  m_index : Inport
  phase : Inport  Port=2
  Clock : Clock
  Constant : Constant  Value=dead_time*f
  Constant2 : Constant  Value=1/f
  Constant4 : Constant
  Data Type Conversion1 : DataTypeConversion
  Data Type Conversion2 : DataTypeConversion
  Gain2 : Gain  Gain=vg_firing
  Gain3 : Gain  Gain=vg_firing
  Gain4 : Gain  Gain=1/2
  Gain5 : Gain  Gain=1/(pi/2)
  Hit Crossing : HitCross  ShowOutputPort=off
  Hit Crossing1 : HitCross  ShowOutputPort=off
  MATLAB Function : MATLAB Function  TreatAsAtomicUnit=on
  Relational Operator1 : RelationalOperator  Operator=<=  InputSameDT=off
  Relational Operator2 : RelationalOperator  Operator=<=  InputSameDT=off
  Saturation1 : Saturate  UpperLimit=m_up  LowerLimit=m_low
  Sum : Sum  Inputs=|++  SaturateOnIntegerOverflow=on
  Sum1 : Sum  Inputs=-+|  SaturateOnIntegerOverflow=on
  Sum3 : Sum  Inputs=|++
  m1 : Outport
  m2 : Outport  Port=2
  wires:
  Relational Operator1/1 -> Data Type Conversion1/1
  m_index/1 -> Saturation1/1
  Relational Operator2/1 -> Data Type Conversion2/1
  Data Type Conversion2/1 -> Gain3/1, Hit Crossing1/1
  Constant/1 -> Sum/2, Sum1/1
  Saturation1/1 -> Sum/1, Sum1/2
  Sum/1 -> Relational Operator1/1
  Sum1/1 -> Relational Operator2/2
  Gain4/1 -> Relational Operator2/1, Relational Operator1/2
  Data Type Conversion1/1 -> Hit Crossing/1, Gain2/1
  Gain2/1 -> m1/1
  Gain3/1 -> m2/1
  Clock/1 -> MATLAB Function/1(t)
  Constant2/1 -> MATLAB Function/3(period)
  phase/1 -> MATLAB Function/2(phase)
  MATLAB Function/1(y) -> Gain5/1
  Gain5/1 -> Sum3/1
  Sum3/1 -> Gain4/1
  Constant4/1 -> Sum3/2

== matlab function im_inv_model/induction motor/control performance evaluation/adc2dq_s_2/alphabeta2xieta ==
  data: alpha input; d output; beta input; theta input; q output
function [d,q] = alphabeta2xieta(alpha,beta,theta)

    d  =  alpha*cos(theta) + beta*sin(theta);
    q = -alpha*sin(theta) + beta*cos(theta);

end

== matlab function im_inv_model/induction motor/control performance evaluation/adc2dq_slip_2/abc2alphabeta ==
  data: abc input; alpha output; beta output
function [alpha,beta] = abc2alphabeta(abc)

alpha = 2/3*(abc(1) - 1/2*abc(2) - 1/2*abc(3));
beta  = 1/sqrt(3)*(abc(2) - abc(3));

end

== matlab function im_inv_model/induction motor/control performance evaluation/adc2dq_slip_2/alphabeta2xieta ==
  data: alpha input; d output; beta input; theta input; q output
function [d,q] = alphabeta2xieta(alpha,beta,theta)

    d  =  alpha*cos(theta) + beta*sin(theta);
    q = -alpha*sin(theta) + beta*cos(theta);

end

== matlab function im_inv_model/inverter//ctrl/im_ctrl/im_control/data_analysis/double_integrator_observer_2/bounder1 ==
  data: u input; y output
function y = bounder(u)
    
    y = -pi + mod(u+3*pi,2*pi);
end

== matlab function im_inv_model/inverter//ctrl/im_ctrl/im_control/data_analysis/double_integrator_observer_2/bounder2 ==
  data: u input; y output
function y = bounder(u)
    
    y = -pi + mod(u+3*pi,2*pi);
end

== matlab function im_inv_model/inverter//ctrl/inverter/inverter/three phase pwm1/uvw2alphabeta1 ==
  data: alpha input; u output; beta input; v output; w output
function [u,v,w] = alphabeta2uvw(alpha,beta)

u  = alpha;
v  = -0.5*alpha+sqrt(3)/2*beta;
w  = -0.5*alpha-sqrt(3)/2*beta;

end

== matlab function im_inv_model/inverter//ctrl/im_ctrl/im_control/data_analysis/double_integrator_observer_3/bounder1 ==
  data: u input; y output
function y = bounder(u)
    
    y = -pi + mod(u+3*pi,2*pi);
end

== matlab function im_inv_model/inverter//ctrl/im_ctrl/im_control/data_analysis/double_integrator_observer_3/bounder2 ==
  data: u input; y output
function y = bounder(u)
    
    y = -pi + mod(u+3*pi,2*pi);
end

== matlab function im_inv_model/inverter//ctrl/im_ctrl/im_control/u//f control/uf_phase_generation/bounder ==
  data: u input; y output
function y = bounder(u)
    
    u = -pi + mod(u+3*pi,2*pi);
    
    y = u;
end

== matlab function im_inv_model/induction motor/mechanical data/double_integrator_observer_for_im/bounder1 ==
  data: u input; y output
function y = bounder(u)
    y = -pi + mod(u+3*pi,2*pi);
end

== matlab function im_inv_model/inverter//ctrl/im_ctrl/im_control/data_analysis/double_integrator_observer_1/bounder2 ==
  data: u input; y output
function y = bounder(u)
    
    y = -pi + mod(u+3*pi,2*pi);
end

== matlab function im_inv_model/induction motor/mechanical data/encoder_measure/bounder2 ==
  data: u input; y output
function y = bounder(u) 
    y = -pi + mod(u+3*pi,2*pi);
end

== matlab function im_inv_model/inverter//ctrl/inverter/inverter/sv_pwm/modulator1/PWM generator 2/MATLAB Function ==
  data: t input; y output; phase input; period input
function y = trgo(t,phase,period)
x = sin(2*pi/period*t - phase -pi/2);
y = asin(x);

== matlab function im_inv_model/inverter//ctrl/inverter/inverter/sv_pwm/modulator1/PWM generator 3/MATLAB Function ==
  data: t input; y output; phase input; period input
function y = trgo(t,phase,period)
x = sin(2*pi/period*t - phase -pi/2);
y = asin(x);

== matlab function im_inv_model/inverter//ctrl/im_ctrl/im_control/flux_estimator/bounder3 ==
  data: u input; y output
function y = bounder(u)
    
    y = -pi + mod(u+3*pi,2*pi);
    
end

== matlab function im_inv_model/inverter//ctrl/im_ctrl/im_control/data_analysis/double_integrator_observer_1/bounder1 ==
  data: u input; y output
function y = bounder(u)
    
    y = -pi + mod(u+3*pi,2*pi);
end

== matlab function im_inv_model/inverter//ctrl/im_ctrl/im_control/flux_estimator/bounder1 ==
  data: u input; y output
function y = bounder(u)
    
    y = -pi + mod(u+3*pi,2*pi);
    
end

== matlab function im_inv_model/inverter//ctrl/inverter/inverter/sv_pwm/modulator1/PWM generator 1/MATLAB Function ==
  data: t input; y output; phase input; period input
function y = trgo(t,phase,period)
x = sin(2*pi/period*t - phase -pi/2);
y = asin(x);

== matlab function im_inv_model/induction motor/control performance evaluation/adc2dq_s_1/abc2alphabeta ==
  data: abc input; alpha output; beta output
function [alpha,beta] = abc2alphabeta(abc)

alpha = 2/3*(abc(1) - 1/2*abc(2) - 1/2*abc(3));
beta  = 1/sqrt(3)*(abc(2) - abc(3));

end

== matlab function im_inv_model/inverter//ctrl/inverter/inverter/three phase pwm/modulator/PWM generator 1/MATLAB Function ==
  data: t input; y output; phase input; period input
function y = trgo(t,phase,period)
x = sin(2*pi/period*t - phase);
y = asin(x);

== matlab function im_inv_model/inverter//ctrl/inverter/inverter/three phase pwm/uvw2alphabeta1 ==
  data: alpha input; u output; beta input; v output; w output
function [u,v,w] = alphabeta2uvw(alpha,beta)

u  = alpha;
v  = -0.5*alpha+sqrt(3)/2*beta;
w  = -0.5*alpha-sqrt(3)/2*beta;

end

== matlab function im_inv_model/induction motor/mechanical data/double_integrator_observer_for_im/bounder2 ==
  data: u input; y output
function y = bounder(u)
    y = -pi + mod(u+3*pi,2*pi);
end

== matlab function im_inv_model/inverter//ctrl/inverter/inverter/three phase pwm/modulator/PWM generator 2/MATLAB Function ==
  data: t input; y output; phase input; period input
function y = trgo(t,phase,period)
x = sin(2*pi/period*t - phase);
y = asin(x);

== matlab function im_inv_model/inverter//ctrl/inverter/inverter/three phase pwm/modulator/PWM generator 3/MATLAB Function ==
  data: t input; y output; phase input; period input
function y = trgo(t,phase,period)
x = sin(2*pi/period*t - phase);
y = asin(x);

== matlab function im_inv_model/induction motor/control performance evaluation/adc2dq_slip_1/abc2alphabeta ==
  data: abc input; alpha output; beta output
function [alpha,beta] = abc2alphabeta(abc)

alpha = 2/3*(abc(1) - 1/2*abc(2) - 1/2*abc(3));
beta  = 1/sqrt(3)*(abc(2) - abc(3));

end

== matlab function im_inv_model/induction motor/control performance evaluation/adc2dq_slip_1/alphabeta2xieta ==
  data: alpha input; d output; beta input; theta input; q output
function [d,q] = alphabeta2xieta(alpha,beta,theta)

    d  =  alpha*cos(theta) + beta*sin(theta);
    q = -alpha*sin(theta) + beta*cos(theta);

end

== matlab function im_inv_model/induction motor/control performance evaluation/adc2dq_s_2/abc2alphabeta ==
  data: abc input; alpha output; beta output
function [alpha,beta] = abc2alphabeta(abc)

alpha = 2/3*(abc(1) - 1/2*abc(2) - 1/2*abc(3));
beta  = 1/sqrt(3)*(abc(2) - abc(3));

end

== matlab function im_inv_model/induction motor/control performance evaluation/adc2dq_s_1/alphabeta2xieta ==
  data: alpha input; d output; beta input; theta input; q output
function [d,q] = alphabeta2xieta(alpha,beta,theta)

    d  =  alpha*cos(theta) + beta*sin(theta);
    q = -alpha*sin(theta) + beta*cos(theta);

end
